simulink model "ATOM_parking_chain"  (R2026a)
settings: Solver=ode4  StopTime=100  FixedStep=0.01
StopFcn:
  | % Put every new figure in the same MATLAB Figures window as a docked tab.
  | set(groot, 'defaultFigureWindowStyle', 'docked');
  | 
  | if exist('costmap_active', 'var') && ...
  |         exist('vehicle', 'var') && ...
  |         exist('parking_path', 'var') && ...
  |         ~isempty(parking_path)
  | 
  |     plotPlan(costmap_active, vehicle, parking_path);
  | 
  | else
  | 
  |     warning('No valid parking path is available for plotting.');
  | 
  | end
  | 
  | PlotControllerReferences( ...
  |     out.controller_reference_log);
  | 
  | PlotControllerTracking( ...
  |     out.controller_tracking_log);
undefined symbols (not defined in the file): lateral, longitudinal, stanley, vehicle
(part 4 of 11)

== matlab function ATOM_parking_chain/Subsystem1/parkingNMPC ==
  settings: updateMethod=DISCRETE  sampleTime=0.04
  data: tx input; path_length output; ty input; tqz input; tqw input; tdf input; tdr input; tvx input; tax input; max_q output; X input; Y input; s_now output; ey_now output; qz input; qw input; vx input; ax_meas input; df input; dr input; x_now output; veh input; longitudinal_mode output; df_rate_cmd output; dr_rate_cmd output; nmpc_info output; segment_done output; active_segment input; endpoint_error output; a_cmd_history input; costmap input; df_ref_out output; dr_ref_out output; t_ref input; s_ref input; x_ref input; y_ref input; psi_ref input; v_ref input; a_ref input; df_nom input; dr_nom input
function [path_length, max_q, s_now, ey_now, x_now, ...
    longitudinal_mode, df_rate_cmd, dr_rate_cmd, nmpc_info, ...
    segment_done, endpoint_error, ...
    df_ref_out, dr_ref_out] = parkingNMPC( ...
    tx,ty,tqz,tqw,tdf,tdr,tvx,tax, ...
    X,Y,qz,qw,vx,ax_meas,df,dr,veh, ...
    active_segment,a_cmd_history,costmap,t_ref,s_ref,x_ref,y_ref,psi_ref,v_ref,a_ref,df_nom,dr_nom)
% Steering-only NMPC: U(:,1:2) are front/rear steering-rate commands.
% The separate parkingLongitudinalController provides acceleration.
% Both prediction loops reproduce its feedforward-plus-P law.
% Expected timing: controller/prediction 0.04 s, steering delay 0.24 s,
% acceleration delay 0.10 s. a_cmd_history is a 3-by-1 vector containing
% the actual pre-transport-delay acceleration commands, oldest first.
% This version has 13 outputs, matching the supplied Subsystem1 wiring.
persistent ref s_prev U_prev buf terminal_creep_steps
persistent previous_active_segment
persistent steering_command_state
persistent steering_alignment_pending

N  = 15;
nd = 6;

if isempty(previous_active_segment)
    previous_active_segment = active_segment;
    segment_changed = false;
else
    segment_changed = ...
        active_segment ~= previous_active_segment;

    previous_active_segment = active_segment;
end

% Build the reference during the first execution.
if isempty(ref)
    ref = buildRef( ...
    t_ref,s_ref,x_ref,y_ref,psi_ref,v_ref,a_ref, ...    
    df_nom,dr_nom);
end

if isempty(s_prev)
    s_prev = 0;
end

if isempty(U_prev)
    % Columns: front steering rate, rear steering rate
    U_prev = zeros(N,2);
end

if isempty(buf)
    % Initialize the delayed-command history from the measured wheel angles.
    buf = repmat([df, dr], nd, 1);
end

if isempty(steering_command_state)
    steering_command_state = [df,dr];
end

% History of acceleration commands already sent to the vehicle.
% Three samples are retained because the acceleration delay is 0.10 s,
% equivalent to 2.5 controller intervals at Ts = 0.04 s.
% Acceleration commands sampled externally every 0.04 seconds.
aBuf = a_cmd_history;

if isempty(terminal_creep_steps)
    terminal_creep_steps = 0.0;
end

if isempty(steering_alignment_pending)
    steering_alignment_pending = true;
end

% Rebuild the reference once when the segment changes.
if logical(segment_changed)
    ref = buildRef( ...
    t_ref,s_ref,x_ref,y_ref,psi_ref,v_ref,a_ref, ...
    df_nom,dr_nom);
    s_prev = 0;
    % Columns: front steering rate, rear steering rate
    U_prev = zeros(N,2);
    terminal_creep_steps = 0.0;
    steering_alignment_pending = true;

end
path_length = ref.s(end); max_q = max(ref.q);
[s_new, ey_now] = whereOnPath(ref, X, Y, s_prev);
s_now  = min(max(s_new, s_prev), s_prev + 0.5);   % never backwards, never a big jump forward

df_ref_out = lookupS(ref.s, ref.df, s_now);
dr_ref_out = lookupS(ref.s, ref.dr, s_now);

s_prev = s_now;

% --- the state of the car right now ---
psi   = 2*atan2(qz, qw);
x_now = [X; Y; psi; vx; df; dr; ax_meas]; %state of the nmpc controller
P     = carNumbers(veh);
M = mapNumbers(costmap);
current_collision_constraint = ...
    poseCollisionConstraint(X,Y,psi,P,M);

% Remaining path distance used by the maneuver supervisor.
d_left = max(ref.s(end) - s_now, 0);

% The segment is complete only after reaching its end and stopping.
% Actual distance from the vehicle's rear axle to the segment endpoint.
endpoint_distance = hypot( ...
    X - ref.X(end), ...
    Y - ref.Y(end));

% Heading error relative to the segment endpoint, wrapped to [-pi, pi].
heading_difference = psi - ref.psi(end);

endpoint_heading_error = atan2( ...
    sin(heading_difference), ...
    cos(heading_difference));

% ---------------- Segment arrival and stop supervision ----------------
%
% Precise tolerance:
% Used to evaluate the final tracking quality.
%
% Arrival tolerance:
% Used to decide whether the stopped vehicle may proceed to the next
% forward/reverse segment.

end_distance_tolerance = 0.05;       % [m]
end_heading_tolerance  = 2*pi/180;   % [rad]

arrive_distance_tolerance = 0.20;       % [m]
arrive_heading_tolerance = 5*pi/180;   % [rad]

stop_speed_tolerance = 0.02;         % [m/s]

% Because s_now is not allowed to decrease, end_reached remains true
% after the vehicle reaches the final path progress.
end_reached = ...
    d_left <= 0.02;

% High-accuracy endpoint condition.
pose_acceptable = ...
    (endpoint_distance <= end_distance_tolerance) && ...
    (abs(endpoint_heading_error) <= end_heading_tolerance);

% Practical condition for authorizing the next gear segment.
pose_arrived = ...
    (endpoint_distance <= arrive_distance_tolerance) && ...
    (abs(endpoint_heading_error) <= arrive_heading_tolerance);

% The vehicle must be nearly stationary before changing segments.
stopped = ...
    abs(vx) <= stop_speed_tolerance;

% Steering must be positioned for the new segment before motion begins.
steering_alignment_tolerance = 2*pi/180;

segment_start_front_steering = ref.df(1);
segment_start_rear_steering  = ref.dr(1);

front_steering_aligned = ...
    abs(df-segment_start_front_steering) <= ...
    steering_alignment_tolerance;

rear_steering_aligned = ...
    abs(dr-segment_start_rear_steering) <= ...
    steering_alignment_tolerance;

steering_aligned = ...
    front_steering_aligned && ...
    rear_steering_aligned;

% Release the alignment hold only after the measured wheels—not merely the
% requested commands—have reached the new segment's starting angles.
if steering_alignment_pending && stopped && steering_aligned
    steering_alignment_pending = false;
end

steering_alignment_active = steering_alignment_pending;

% Advance to the next segment only after reaching the endpoint progress,
% stopping, and satisfying the practical arrival tolerance.
segment_done = ...
    end_reached && ...
    stopped && ...
    pose_arrived;

% If the vehicle stops outside the arrival tolerance, keep the current
% segment active and report the failure through the controller status.
arrival_failed = ...
    end_reached && ...
    stopped && ...
    ~pose_arrived;

% Permanent endpoint diagnostics:
%   element 1: position error [m]
%   element 2: signed heading error [deg]
endpoint_error = [ ...
    endpoint_distance; ...
    endpoint_heading_error*180/pi];

% Longitudinal modes:
%   0 = follow the planned velocity profile
%   1 = slow terminal approach
%   2 = stop


longitudinal_mode = 0.0;

if steering_alignment_active

    % Keep the vehicle stopped while the wheels align.
    longitudinal_mode = 2.0;

elseif end_reached

    if pose_arrived
        % Correct endpoint pose reached.
        longitudinal_mode = 2.0;
    else
        % Continue slowly to correct the endpoint pose.
        longitudinal_mode = 1.0;
    end

end

% --- steering ---
use_nmpc = true;      % false = D1 baseline (follow the plan blindly)
% [X error, Y error, heading error, nominal steering, command change]
% Velocity/acceleration remain predicted states but have no cost terms
% in this five-weight steering objective.
w = [10, 10, 1, 0.1, 0.1];

if use_nmpc
    x0   = x_now;                                          % start from the real car
    cost = @(u) score( ...
        reshape(u,N,2), ...
        x0, ...
        s_now, ...
        buf, ...
        steering_command_state, ...
        aBuf, ...
        ref, ...
        P, ...
        w, ...
        longitudinal_mode);

    nonlinear_constraint = @(u) collisionConstraints( ...
        u, ...
        x0, ...
        s_now, ...
        buf, ...
        steering_command_state, ...
        aBuf, ...
        ref, ...
        P, ...
        M, ...
        longitudinal_mode);

    lb = -P.rateLim*ones(2*N,1);
    ub =  P.rateLim*ones(2*N,1);
    % Shared tolerance for the optimizer and the independent collision check.
    collision_tolerance = 1e-6;
    
    opts = optimoptions('fmincon', ...
        'Algorithm', 'sqp', ...
        'Display', 'none', ...
        'MaxIterations', 30, ...
        'ConstraintTolerance', collision_tolerance);
    solve_start = tic;
    
    % Optimize the front and rear steering commands.
    % Steering-angle limits are hard constraints.
    % Command changes are discouraged by the dU term in the cost function.
    [u, J_best, flag, solver_output] = fmincon( ...
        cost, U_prev(:), ...
        [], [], [], [], ...
        lb, ub, ...
        nonlinear_constraint, opts);
    
    solve_time = toc(solve_start);
    % Check whether the returned cost and commands are finite.
    finite_solution = ...
        isfinite(J_best) && ...
        all(isfinite(u));

    % Small tolerance for numerical round-off at the steering limits.
    bound_tolerance = 1e-9;

    % Check whether all optimized commands respect their bounds.
    inside_bounds = ...
        all(u >= lb - bound_tolerance) && ...
        all(u <= ub + bound_tolerance);

    % Verify the nonlinear collision constraints independently after
    % fmincon returns its candidate solution.
    collision_feasible = false;

    % Do not evaluate geometric constraints using nonfinite commands or
    % a candidate already declared invalid by the solver.
    if finite_solution && flag >= 0

        [candidate_collision_constraints,~] = ...
            collisionConstraints( ...
            u, ...
            x0, ...
            s_now, ...
            buf, ...
            steering_command_state,...
            aBuf, ...
            ref, ...
            P, ...
            M, ...
            longitudinal_mode);

        collision_feasible = ...
            all(isfinite(candidate_collision_constraints)) && ...
            all(candidate_collision_constraints <= ...
            collision_tolerance);
    end


    % Classify the optimization result.
    if ~finite_solution || ...
       ~inside_bounds || ...
       ~collision_feasible || ...
       flag < 0

        % The optimizer returned an unusable result.
        controller_status = 2;

    elseif flag == 0 || solve_time > P.controlTs

        % The result is usable, but the solver did not converge normally
        % or exceeded the controller sampling period.
        controller_status = 1;

    else

        % The solver returned a normal valid result.
        controller_status = 0;

    end

    % Endpoint-arrival diagnostics.
    % Preserve status 2 when the optimizer result itself is invalid.
    %
    % Status 5:
    %   stopped outside the 0.20 m / 5 degree arrival tolerance.
    %
    % Status 4:
    %   segment accepted using the arrival tolerance, but outside the
    %   more precise 0.05 m / 2 degree quality tolerance.
    
    if controller_status ~= 2
    
        if arrival_failed
            controller_status = 5;
    
        elseif segment_done && ~pose_acceptable
            controller_status = 4;
        end
    
    end
        
    % If the new optimizer result is unusable, verify whether the
    % remaining previous steering plan is still safe from the current
    % measured state and with the current costmap.
    fallback_collision_feasible = false;

    if controller_status == 2

        fallback_u = U_prev(:);

        fallback_finite = ...
            all(isfinite(fallback_u));

        fallback_inside_bounds = ...
            all(fallback_u >= lb - bound_tolerance) && ...
            all(fallback_u <= ub + bound_tolerance);

        if fallback_finite && fallback_inside_bounds

            [fallback_collision_constraints,~] = ...
                collisionConstraints( ...
                fallback_u, ...
                x0, ...
                s_now, ...
                buf, ...
                steering_command_state,...
                aBuf, ...
                ref, ...
                P, ...
                M, ...
                longitudinal_mode);

            fallback_collision_feasible = ...
                all(isfinite(fallback_collision_constraints)) && ...
                all(fallback_collision_constraints <= ...
                collision_tolerance);
        end
    end

    % Convert the new optimizer result into an N-by-2 steering plan.
    U_candidate = reshape(u, N, 2);
    
    % Select the steering plan that the controller is allowed to use.
    if controller_status == 2

        if fallback_collision_feasible

            % The new result is unusable, but the remaining previous
            % plan is still collision-free from the current state.
            U_selected = U_prev;

        else

            % Neither the new solution nor the previous plan is safe.
            % Request braking from the separate longitudinal controller.
            longitudinal_mode = 2.0;

            % Hold the current measured steering angles while stopping.
            % Move the desired steering command toward the measured wheel angles.
            target_front_angle = max( ...
                -P.steerMax, ...
                min(P.steerMax,df));
            
            target_rear_angle = max( ...
                -P.steerMax, ...
                min(P.steerMax,dr));
            
            hold_front_rate = ...
                (target_front_angle-steering_command_state(1))/P.controlTs;
            
            hold_rear_rate = ...
                (target_rear_angle-steering_command_state(2))/P.controlTs;
            
            hold_front_rate = max( ...
                -P.rateLim, ...
                min(P.rateLim,hold_front_rate));
            
            hold_rear_rate = max( ...
                -P.rateLim, ...
                min(P.rateLim,hold_rear_rate));
            
            U_selected = zeros(N,2);
            U_selected(1,1:2) = [hold_front_rate,hold_rear_rate];
            % Status 6 means emergency stop caused by the absence of a
            % collision-feasible steering sequence.
            controller_status = 6;
        end

    else
    
        % Status 0: normal solution.
        % Status 1: degraded but numerically valid solution.
        U_selected = U_candidate;
    
    end

    % Align the wheels directly while the vehicle is stopped at a gear change.
    % This does not move the vehicle body.
    % While steering alignment is pending, keep the vehicle stopped and do
    % not allow the NMPC steering solution to compete with the alignment.
    if steering_alignment_active

        longitudinal_mode = 2.0;
        controller_status = 7;

        % Zero rate holds the current desired steering angles while the
        % vehicle is still coming to rest.
        U_selected = zeros(N,2);

        % Begin changing the steering only after the vehicle has stopped.
        if stopped

            target_front_angle = max( ...
                -P.steerMax, ...
                min(P.steerMax,segment_start_front_steering));

            target_rear_angle = max( ...
                -P.steerMax, ...
                min(P.steerMax,segment_start_rear_steering));

            alignment_front_rate = ...
                (target_front_angle-steering_command_state(1))/P.controlTs;

            alignment_rear_rate = ...
                (target_rear_angle-steering_command_state(2))/P.controlTs;

            alignment_front_rate = max( ...
                -P.rateLim, ...
                min(P.rateLim,alignment_front_rate));

            alignment_rear_rate = max( ...
                -P.rateLim, ...
                min(P.rateLim,alignment_rear_rate));

            U_selected(1,1:2) = ...
                [alignment_front_rate,alignment_rear_rate];
        end
    end

    selected_input = U_selected(1,:);
    
    df_rate_cmd = selected_input(1);
    dr_rate_cmd = selected_input(2);
    
    selected_rate = selected_input(1:2);
    
    % Mirror the external rate-to-angle integrator inside the NMPC.
    
    sent_angle_trajectory = expandSteeringRatePlan( ...
        selected_rate,steering_command_state,P);
    
    steering_command_state = ...
        sent_angle_trajectory(end,:);
    
    updated_delay_history = ...
        [buf;sent_angle_trajectory];
    
    buf = updated_delay_history(end-nd+1:end,:);
    
    % The warm start continues to contain steering rates.
    U_prev = [U_selected(2:end,:);U_selected(end,:)];
    % Status 7 means the vehicle is intentionally stationary while its
    % measured steering aligns with the new segment.
    if steering_alignment_active && ...
            (controller_status == 0 || controller_status == 1)

        controller_status = 7;
    end

    % Status 8:
    % Terminal creep is collision-infeasible, but the stopped vehicle is
    % currently collision-free and sufficiently close to the cusp.
    % Authorize the gear change so the next segment can move away from
    % the obstacle instead of repeating an impossible creep forever.

    cusp_recovery_distance_tolerance = 0.25;        % [m]
    cusp_recovery_heading_tolerance  = 10*pi/180;   % [rad]

    safe_cusp_handoff = ...
        (controller_status == 6) && ...
        arrival_failed && ...
        ~steering_alignment_active && ...
        (current_collision_constraint <= collision_tolerance) && ...
        (endpoint_distance <= cusp_recovery_distance_tolerance) && ...
        (abs(endpoint_heading_error) <= ...
        cusp_recovery_heading_tolerance);

    if safe_cusp_handoff
        segment_done = true;
        controller_status = 8;
    end
    
    nmpc_info = [ ...
        double(J_best); ...
        double(flag); ...
        double(solve_time); ...
        double(solver_output.iterations); ...
        double(solver_output.funcCount); ...
        double(controller_status)];
    % nmpc_info = [ ...
    %     double(current_collision_constraint); ...
    %     double(flag); ...
    %     double(solve_time); ...
    %     double(solver_output.iterations); ...
    %     double(solver_output.funcCount); ...
    %     double(controller_status)];
else
    % Planner steering angles used by the non-NMPC baseline.
    target_front_angle = lookupS(ref.s,ref.df,s_now);
    target_rear_angle  = lookupS(ref.s,ref.dr,s_now);

    % Convert the required angle changes into steering-rate commands.
    df_rate_cmd = ...
        (target_front_angle-steering_command_state(1))/P.controlTs;

    dr_rate_cmd = ...
        (target_rear_angle-steering_command_state(2))/P.controlTs;

    % Apply the same steering-rate limits used by the NMPC.
    df_rate_cmd = max(-P.rateLim,min(P.rateLim,df_rate_cmd));
    dr_rate_cmd = max(-P.rateLim,min(P.rateLim,dr_rate_cmd));

    % Mirror the steering command actually selected in baseline mode.
    selected_rate = [df_rate_cmd,dr_rate_cmd];
    
    sent_angle_trajectory = expandSteeringRatePlan( ...
        selected_rate,steering_command_state,P);
    
    steering_command_state = sent_angle_trajectory(end,:);
    
    updated_delay_history = [buf;sent_angle_trajectory];
    buf = updated_delay_history(end-nd+1:end,:);
    

    U_prev = zeros(N,2);
    
    nmpc_info = [0; 0; 0; 0; 0; 3];
end
end

%--------------------------------------------------------------------------
function P = carNumbers(veh)
% All fields must be created before the structure is read.

collisionMargin = 0.5;

% Controller and internal prediction timing.
controlTs    = 0.04;
predictionTs = 0.04;

P.L        = veh(3);
P.steerMax = veh(10);
P.aMax     = veh(16);
P.rateLim  = veh(18);
P.tau      = veh(22);


%!!!!!!!!!!!!!!!!!!!!!!!!!!!!!!!!!!!!!!!!!!!!!!!!!!!!!!!!!!!!!!!!!!!!!!!!!!
P.vMax = veh(15);       % Prediction clip
P.vStateMax = veh(15);  % Explicit NMPC velocity constraint
%We have considered the maximum velocity in both the prediction and nmpc to
%be equal to the parameter's maximum value although currently it is equal
%to 50m/s!!!!!!!!!!!!!!!!!!!!!!!!!!!!!!!!!!!!!!!!!
%!!!!!!!!!!!!!!!!!!!!!!!!!!!!!!!!!!!!!!!!!!!!!!!!!!!!!!!!!!!!!!!!!!!!!!!!!!

P.controlTs = controlTs;
P.predictionTs = predictionTs;
P.substepsPerControl = round( ...
    controlTs/predictionTs);

P.accDelay = veh(19);
P.accTau   = veh(20);
P.aCmdMax  = 1.0; % Match a_cmd_limit in parkingLongitudinalController.

P.footprintMargin = collisionMargin;

P.footprintBack = ...
    -(veh(6) + collisionMargin/2);

P.footprintFront = ...
    veh(3) + veh(5) + collisionMargin/2;

P.footprintHalfWidth = ...
    (veh(4) + veh(7) + veh(8) + collisionMargin)/2;
end

%--------------------------------------------------------------------------
function M = mapNumbers(costmap)

resolution = double(costmap.info.resolution);

M.res = resolution;
M.width = double(costmap.info.width);
M.height = double(costmap.info.height);

M.originX = double(costmap.info.origin.position.x);
M.originY = double(costmap.info.origin.position.y);

M.grid = double(costmap.data)/100;

M.cellHalf = resolution/2;
end

%--------------------------------------------------------------------------
function [x1,aBuf1,df_raw,dr_raw,vx_raw] = predictStep( ...
    x0,aBuf,aCmd,dfc,drc,P)
% Predict the vehicle over one 0.04 s controller interval.

X   = x0(1);
Y   = x0(2);
psi = x0(3);
vx  = x0(4);
df  = x0(5);
dr  = x0(6);
ax  = x0(7);

%% Steering actuator

ddf = max( ...
    -P.rateLim, ...
    min(P.rateLim,(dfc-df)/P.tau));

ddr = max( ...
    -P.rateLim, ...
    min(P.rateLim,(drc-dr)/P.tau));

df_raw = df + P.predictionTs*ddf;
dr_raw = dr + P.predictionTs*ddr;

df1 = max(-P.steerMax,min(P.steerMax,df_raw));
dr1 = max(-P.steerMax,min(P.steerMax,dr_raw));

%% Acceleration delay and actuator lag

% The 0.04 s interval is divided into two 0.02 s parts.
h = 0.5*P.predictionTs;

% For a 0.10 s transport delay, the delayed command changes halfway
% through the current 0.04 s interval.
aDelayedFirst  = aBuf(1);
aDelayedSecond = aBuf(2);

% First half of the acceleration-actuator response.
axHalf = ax + ...
    h*(aDelayedFirst-ax)/P.accTau;

axHalf = max( ...
    -P.aMax, ...
    min(P.aMax,axHalf));

% Second half of the acceleration-actuator response.
ax1 = axHalf + ...
    h*(aDelayedSecond-axHalf)/P.accTau;

ax1 = max( ...
    -P.aMax, ...
    min(P.aMax,ax1));

% Integrate longitudinal acceleration over the two half-steps.
deltaVFirst = ...
    0.5*h*(ax+axHalf);

deltaVSecond = ...
    0.5*h*(axHalf+ax1);

vxFromAcceleration = ...
    vx + deltaVFirst + deltaVSecond;

% Steering changes during this controller interval, so use its
% midpoint value when predicting the vehicle motion.
dfMid = 0.5*(df+df1);
drMid = 0.5*(dr+dr1);

% Match the longitudinal-velocity equation used by Vehicle_Model.
vxMidForCoupling = ...
    0.5*(vx+vxFromAcceleration);

vehicleSpeedMid = ...
    vxMidForCoupling/max(cos(drMid),0.1);

yawRateMid = ...
    (vxMidForCoupling/P.L) * ...
    (tan(dfMid)-tan(drMid));

rearSteeringVelocityTerm = ...
    yawRateMid*vehicleSpeedMid*sin(drMid);

% Preserve the unconstrained prediction for the optimizer constraint.
vx_raw = vxFromAcceleration + ...
         P.predictionTs*rearSteeringVelocityTerm;

% Keep the numerical guard for state propagation.
vx1 = max(-P.vMax,min(P.vMax,vx_raw));

% Store the acceleration command predicted for the current cycle.
aBuf1 = [aBuf(2:end); aCmd];

%% Vehicle motion

vxMid = 0.5*(vx+vx1);

dRear = ...
    vxMid*P.predictionTs/max(cos(drMid),0.1);

[X1,Y1,psi1] = bicycleGetPose( ...
    X,Y,psi,dfMid,drMid,P.L,dRear);


x1 = [X1;Y1;psi1;vx1;df1;dr1;ax1];


end
%-------------------------------------------------------------------------
function angle_commands = expandSteeringRatePlan( ...
    rate_commands,initial_angle_command,P)

number_of_rate_commands = size(rate_commands,1);
substeps_per_command = P.substepsPerControl;

number_of_angle_samples = ...
    number_of_rate_commands*substeps_per_command;

angle_commands = zeros(number_of_angle_samples,2);

front_command = initial_angle_command(1);
rear_command  = initial_angle_command(2);

sample_index = 0;

for k = 1:number_of_rate_commands

    front_rate = max( ...
        -P.rateLim, ...
        min(P.rateLim,rate_commands(k,1)));

    rear_rate = max( ...
        -P.rateLim, ...
        min(P.rateLim,rate_commands(k,2)));

    for j = 1:substeps_per_command

        front_command = max( ...
            -P.steerMax, ...
            min(P.steerMax, ...
            front_command + ...
            P.predictionTs*front_rate));

        rear_command = max( ...
            -P.steerMax, ...
            min(P.steerMax, ...
            rear_command + ...
            P.predictionTs*rear_rate));

        sample_index = sample_index + 1;

        angle_commands(sample_index,1) = front_command;
        angle_commands(sample_index,2) = rear_command;
    end
end
end

%--------------------------------------------------------------------------
function J = score( ...
    U,x0,s0,buf,steering_command_state, ...
    aBuf,ref,P,w,longitudinal_mode)

% The two optimized inputs are front and rear steering rates.
steering_rate_plan = U(:,1:2);

candidate_angle_commands = expandSteeringRatePlan( ...
    steering_rate_plan,steering_command_state,P);

% Steering commands already waiting in the delay act first.
Ucmd = [buf;candidate_angle_commands];

x = x0;
s = s0;
J = 0;

aBufPrediction = aBuf;
modePrediction = longitudinal_mode;

% Anchor reference time at the current path progress.
t_start = lookupS(ref.s,ref.t,s0);

for k = 1:size(Ucmd,1)

    dLeftPrediction = max(ref.s(end)-s,0.0);

    if dLeftPrediction <= 0.02 && modePrediction ~= 1.0
        modePrediction = 2.0;
    end

    % Predict the external feedforward-plus-P controller at this state.
    % Use the same longitudinal prediction in collisionConstraints.
    aCmdPrediction = longitudinalCommandPrediction( ...
        ref,s,x(4),modePrediction,P);

    [x,aBufPrediction] = predictStep( ...
        x,aBufPrediction,aCmdPrediction, ...
        Ucmd(k,1),Ucmd(k,2),P);

    [s,~] = whereOnPath(ref,x(1),x(2),s);

    t_target = min( ...
        t_start + k*P.predictionTs,ref.t(end));

    X_target = lookupS(ref.t,ref.X,t_target);
    Y_target = lookupS(ref.t,ref.Y,t_target);
    psi_target = lookupS(ref.t,ref.psi,t_target);

    df_target = lookupS(ref.t,ref.df,t_target);
    dr_target = lookupS(ref.t,ref.dr,t_target);

    eX = x(1)-X_target;
    eY = x(2)-Y_target;

    dpsi = x(3)-psi_target;
    epsi = atan2(sin(dpsi),cos(dpsi));

    edf = x(5)-df_target;
    edr = x(6)-dr_target;

    J = J + ...
        w(1)*eX^2 + ...
        w(2)*eY^2 + ...
        w(3)*epsi^2 + ...
        w(4)*(edf^2 + edr^2);
end

% Penalize steering command changes.
steering_angle_changes = P.controlTs*steering_rate_plan;

J = J + w(5)*sum(steering_angle_changes(:).^2);


end

%--------------------------------------------------------------------------
function a_cmd = longitudinalCommandPrediction( ...
    ref, s, vx, longitudinal_mode, P)
% Predict the acceleration command that the separate longitudinal
% controller will generate.

Kp = 1.0;
Kp_stop = 5.0;
terminal_creep_speed = 0.05;

v_ref = lookupS(ref.s,ref.v,s);
a_ref = lookupS(ref.s,ref.a,s);

gear = ref.gear;
Kp_active = Kp;

if longitudinal_mode == 2.0

    % Stop mode.
    v_ref = 0.0;
    a_ref = 0.0;
    Kp_active = Kp_stop;

elseif longitudinal_mode == 1.0

    % Terminal-creep mode.
    v_ref = gear*terminal_creep_speed;
    a_ref = 0.0;

end

speed_error = v_ref-vx;

speed_in_gear = gear*vx;
reference_speed_in_gear = gear*v_ref;
feedforward_in_gear = gear*a_ref;

a_feedforward = a_ref;

% Apply braking feedforward only while the vehicle is moving faster
% than its reference in the intended gear direction.
if feedforward_in_gear < 0.0 && ...
        speed_in_gear <= reference_speed_in_gear

    a_feedforward = 0.0;

end

a_unsaturated = ...
    a_feedforward + Kp_active*speed_error;

a_cmd = max( ...
    -P.aCmdMax, ...
    min(P.aCmdMax,a_unsaturated));

end

%--------------------------------------------------------------------------
function v = lookupS(sv, vv, s)
% Value of vv at distance s along the route (straight line between points).
n = numel(sv);
v = vv(n);
if s <= sv(1), v = vv(1); return; end
if s >= sv(n), return; end
for i = 1:n-1
    if s <= sv(i+1)
        ds = sv(i+1) - sv(i);
        if ds < 1e-12
            v = vv(i+1);
        else
            v = vv(i) + (s - sv(i))/ds*(vv(i+1) - vv(i));
        end
        return;
    end
end
end

%--------------------------------------------------------------------------
function ref = buildRef( ...
    t_ref,s_ref,x_ref,y_ref,psi_ref,v_ref,a_ref, ...
    df_nom,dr_nom)

% Local arrays
t   = t_ref(:);
s   = s_ref(:);
Xr  = x_ref(:);
Yr  = y_ref(:);
psir = psi_ref(:);
vr  = v_ref(:);
ar  = a_ref(:);
dfr = df_nom(:);
drr = dr_nom(:);

n = numel(t);

%% Steering variation per metre

q = zeros(n,1);

for i = 1:n-1

    ds = max(s(i+1)-s(i),1e-9);

    q(i) = max( ...
        abs(dfr(i+1)-dfr(i)), ...
        abs(drr(i+1)-drr(i))) / ds;

end

if n > 1
    q(n) = q(n-1);
else
    q(1) = 0.0;
end

%% Forward or reverse gear

gear = 1;

for i = 1:n

    if abs(vr(i)) > 1e-6
        gear = sign(vr(i));
        break;
    end

end

%% Create every structure field after calculations are complete

ref.t    = t;
ref.s    = s;
ref.X    = Xr;
ref.Y    = Yr;
ref.psi  = psir;
ref.v    = vr;
ref.a    = ar;
ref.df   = dfr;
ref.dr   = drr;
ref.q    = q;
ref.gear = gear;

end

%--------------------------------------------------------------------------
function [s, ey] = whereOnPath(ref, X, Y, s_guess)
% Closest point on the route to (X,Y).
%   s  : how far along the route that point is
%   ey : how far to the side the car is (left positive)
n = numel(ref.s);
best = inf;  s = s_guess;  ey = 0;
win  = 1.5;

for pass = 1:2
    for i = 1:n-1
        if abs(ref.s(i) - s_guess) > win
            continue;
        end
        ax = ref.X(i);   ay = ref.Y(i);
        bx = ref.X(i+1); by = ref.Y(i+1);
        L2 = (bx-ax)^2 + (by-ay)^2;
        t  = ((X-ax)*(bx-ax) + (Y-ay)*(by-ay)) / max(L2, 1e-12);
        t  = min(max(t, 0), 1);
        px = ax + t*(bx-ax);   py = ay + t*(by-ay);
        d2 = (X-px)^2 + (Y-py)^2;
        if d2 < best
            best = d2;
            s  = ref.s(i) + t*(ref.s(i+1) - ref.s(i));
            ey = sign((bx-ax)*(Y-ay) - (by-ay)*(X-ax)) * sqrt(d2);
        end
    end
    if best < inf, break; end
    win = inf;
end
end

%--------------------------------------------------------------------------
function cPose = poseCollisionConstraint(X,Y,psi,P,M) %This function is added in our way for the implementation of the non-linear hard constraint of the obstacle avoidance
% Continuous collision measure for one predicted vehicle pose.
%
% fmincon convention:
%   cPose < 0  : collision-free
%   cPose = 0  : touching the obstacle or map boundary
%   cPose > 0  : collision or map-boundary violation

% Nearby obstacles begin influencing the constraint from this distance.
% This is not an additional vehicle safety margin.
influenceDistance = 1.0;

% Prevent exact geometric touching from being accepted because of
% numerical round-off.
numericalClearance = 1e-4;

ct = cos(psi);
st = sin(psi);

%% Enlarged vehicle rectangle

back = P.footprintBack;
front = P.footprintFront;
halfWidth = P.footprintHalfWidth;

vehicleCentreOffset = 0.5*(front + back);
vehicleHalfLength = 0.5*(front - back);

vehicleCentreX = X + ct*vehicleCentreOffset;
vehicleCentreY = Y + st*vehicleCentreOffset;

% Projection of the rotated vehicle rectangle onto the world axes.
vehicleProjectionX = ...
    vehicleHalfLength*abs(ct) + halfWidth*abs(st);

vehicleProjectionY = ...
    vehicleHalfLength*abs(st) + halfWidth*abs(ct);

vehicleMinX = vehicleCentreX - vehicleProjectionX;
vehicleMaxX = vehicleCentreX + vehicleProjectionX;
vehicleMinY = vehicleCentreY - vehicleProjectionY;
vehicleMaxY = vehicleCentreY + vehicleProjectionY;

%% Map-boundary constraint

mapMinX = M.originX - M.cellHalf;
mapMaxX = M.originX + (M.width-1)*M.res + M.cellHalf;

mapMinY = M.originY - M.cellHalf;
mapMaxY = M.originY + (M.height-1)*M.res + M.cellHalf;

boundaryConstraint = max( ...
    max( ...
        mapMinX - vehicleMinX, ...
        vehicleMaxX - mapMaxX), ...
    max( ...
        mapMinY - vehicleMinY, ...
        vehicleMaxY - mapMaxY));

%% Find nearby costmap cells

searchHalfX = ...
    vehicleProjectionX + M.cellHalf + influenceDistance;

searchHalfY = ...
    vehicleProjectionY + M.cellHalf + influenceDistance;

ix0 = ceil( ...
    (vehicleCentreX-searchHalfX-M.originX)/M.res);

ix1 = floor( ...
    (vehicleCentreX+searchHalfX-M.originX)/M.res);

iy0 = ceil( ...
    (vehicleCentreY-searchHalfY-M.originY)/M.res);

iy1 = floor( ...
    (vehicleCentreY+searchHalfY-M.originY)/M.res);

ix0 = max(0,ix0);
ix1 = min(M.width-1,ix1);

iy0 = max(0,iy0);
iy1 = min(M.height-1,iy1);

% A value of -influenceDistance is safely feasible.
obstacleConstraint = -influenceDistance;

% Projection of a square costmap cell onto either vehicle axis.
cellProjectionRotated = ...
    M.cellHalf*(abs(ct) + abs(st));

%% Rectangle-versus-cell constraints

if ix0 <= ix1 && iy0 <= iy1

    for iy = iy0:iy1
        for ix = ix0:ix1

            cellValue = M.grid(iy+1,ix+1);

            % Occupied cells are >= 1.
            % Unknown cells are negative and are also unsafe.
            if cellValue >= 1.0 || cellValue < 0.0

                cellX = M.originX + ix*M.res;
                cellY = M.originY + iy*M.res;

                dx = cellX - vehicleCentreX;
                dy = cellY - vehicleCentreY;

                % Overlap on the two world axes.
                overlapWorldX = ...
                    vehicleProjectionX + M.cellHalf - abs(dx);

                overlapWorldY = ...
                    vehicleProjectionY + M.cellHalf - abs(dy);

                % Cell position expressed along the vehicle axes.
                distanceLongitudinal = ct*dx + st*dy;
                distanceLateral = -st*dx + ct*dy;

                % Overlap on the two vehicle axes.
                overlapLongitudinal = ...
                    vehicleHalfLength + ...
                    cellProjectionRotated - ...
                    abs(distanceLongitudinal);

                overlapLateral = ...
                    halfWidth + ...
                    cellProjectionRotated - ...
                    abs(distanceLateral);

                % SAT collision measure for this occupied cell.
                cellConstraint = min( ...
                    min(overlapWorldX,overlapWorldY), ...
                    min(overlapLongitudinal,overlapLateral));

                obstacleConstraint = max( ...
                    obstacleConstraint, ...
                    cellConstraint);
            end
        end
    end
end

% The worst condition determines whether this pose is feasible.
cPose = ...
    max(boundaryConstraint,obstacleConstraint) + ...
    numericalClearance;
end

%--------------------------------------------------------------------------
function [c,ceq] = collisionConstraints( ...
    u,x0,s0,buf,steering_command_state, ...
    aBuf,ref,P,M,longitudinal_mode)

N = 15;

% Two optimized steering rates per prediction stage.
U = reshape(u,N,2);

steering_rate_plan = U(:,1:2);


candidate_angle_commands = expandSteeringRatePlan( ...
    steering_rate_plan,steering_command_state,P);

Ucmd = [buf;candidate_angle_commands];

numberOfPredictedSteps = size(Ucmd,1);

% One collision, four steering-angle, and two velocity inequalities.
constraints_per_step = 7;
c = zeros(constraints_per_step*numberOfPredictedSteps,1);
ceq = zeros(0,1);

x = x0;
s = s0;

aBufPrediction = aBuf;
modePrediction = longitudinal_mode;

for k = 1:numberOfPredictedSteps

    dLeftPrediction = max(ref.s(end)-s,0.0);

    if dLeftPrediction <= 0.02 && modePrediction ~= 1.0
        modePrediction = 2.0;
    end

    % Match the feedforward-plus-P prediction used by score.
    aCmdPrediction = longitudinalCommandPrediction( ...
        ref,s,x(4),modePrediction,P);

    [x,aBufPrediction,df_raw,dr_raw,vx_raw] = predictStep( ...
        x,aBufPrediction,aCmdPrediction,Ucmd(k,1),Ucmd(k,2),P);

    [s,~] = whereOnPath(ref,x(1),x(2),s);

    i = constraints_per_step*(k-1);

    c(i+1) = poseCollisionConstraint( ...
        x(1),x(2),x(3),P,M);

    c(i+2) =  df_raw-P.steerMax;
    c(i+3) = -df_raw-P.steerMax;

    c(i+4) =  dr_raw-P.steerMax;
    c(i+5) = -dr_raw-P.steerMax;
    % Hard predicted-velocity state constraint:
    % -P.vStateMax <= vx_raw <= P.vStateMax
    c(i+6) =  vx_raw - P.vStateMax;
    c(i+7) = -vx_raw - P.vStateMax;
end

end

== matlab function ATOM_parking_chain/Vehicle_Model1/Vehicle Dynamics/MATLAB Function ==
  data: state input Bus: VehicleInternalStateBus size=1; d_state output Bus: VehicleInternalStateBus size=1; command input Bus: ControlCMDBus size=1; veh input; rear_steering_command input
function d_state = vehicleDynamics(state, command, veh, rear_steering_command)

%%%%%%%%%%%%%%%%%%%%%%%%%%%%%%%%%%%%%%
%%%%%%%%%%%%%%%%%%%%%%%%%%%%%%%%%%%%%%
% Description:
% This vehicleDynamics model follows DELAY_STEER_ACC_GEARED
% model, it doesn't presents a model for gear management
% since its not something we're going to modify on Autoware for 4WS
% implementation.
%
% Inputs:
% - state: VehicleInternalStateBus. It contains the state of the vehicle
%          at time instant t. 
% - command: /control/command/control_cmd topic --> ControlCMDBus.
%          It contains the desired acc and steering commands coming from
%          the control region.
%
% - Parameters
% - vehicle: vehicle parameters struct defined in vehicleParameters.m.

% Outputs: 
% - d_state: It contains the derivative of the state of the vehicle at time
%          instant t+1.
%%%%%%%%%%%%%%%%%%%%%%%%%%%%%%%%%%%%%%
%%%%%%%%%%%%%%%%%%%%%%%%%%%%%%%%%%%%%%


% inside MATLAB Function: input is veh_in (1xN double)
v = veh; % 1xN numeric row

vehicle.param.wheel_radius    = v(1);
vehicle.param.wheel_width     = v(2);
vehicle.param.wheel_base      = v(3);
vehicle.param.wheel_tread     = v(4);
vehicle.param.front_overhang  = v(5);
vehicle.param.rear_overhang   = v(6);
vehicle.param.left_overhang   = v(7);
vehicle.param.right_overhang  = v(8);
vehicle.param.vehicle_height  = v(9);
vehicle.param.max_steer_angle = v(10);

% decode integer-coded enums (example)
vehicle.sim.vehicle_model_type = int32(v(11));    % or map to strings if needed
vehicle.sim.initialize_source  = int32(v(12));

vehicle.sim.timer_sampling_time_ms = v(13);
vehicle.sim.add_measurement_noise = logical(v(14));
vehicle.sim.vel_lim        = v(15);
vehicle.sim.vel_rate_lim   = v(16);
vehicle.sim.steer_lim      = v(17);
vehicle.sim.steer_rate_lim = v(18);
vehicle.sim.acc_time_delay = v(19);
vehicle.sim.acc_time_constant = v(20);
vehicle.sim.steer_time_delay   = v(21);
vehicle.sim.steer_time_constant= v(22);
vehicle.sim.x_stddev = v(23);
vehicle.sim.y_stddev = v(24);
vehicle.sim.steer_dead_band = v(25);
vehicle.sim.steer_bias = v(26);
vehicle.sim.debug_acc_scaling_factor = v(27);
vehicle.sim.debug_steer_scaling_factor = v(28);

% Parameter for 4WS
vehicle.param.rear_steering_ratio = veh(29);
rear_steering_ratio = vehicle.param.rear_steering_ratio;

%% ==========================
% Saturation function
% ===========================

sat = @(val, upper, lower) min(max(val,lower),upper);



%% ==========================
% Current state
% ===========================

vx = sat( ...
    state.vx,...
    vehicle.sim.vel_lim,...
   -vehicle.sim.vel_lim);


acc = sat( ...
    state.acc,...
    vehicle.sim.vel_rate_lim,...
   -vehicle.sim.vel_rate_lim);


yaw = state.yaw;

steer_front = state.steer_front;
steer_rear = state.steer_rear;          % Modified for 4WS  


%% ==========================
% Input commands
% ===========================

acc_des = sat( ...
    command.longitudinal.acceleration,...
    vehicle.sim.vel_rate_lim,...
   -vehicle.sim.vel_rate_lim);


acc_des = acc_des * ...
    vehicle.sim.debug_acc_scaling_factor;



steer_front_des = sat( ...
    command.lateral.steering_tire_angle,...
    vehicle.sim.steer_lim,...
   -vehicle.sim.steer_lim);


steer_front_des = steer_front_des * ...
    vehicle.sim.debug_steer_scaling_factor;

steer_rear_des = sat( ...                                            % Modified for 4WS
    rear_steering_command,...
    vehicle.sim.steer_lim,...
    -vehicle.sim.steer_lim);


steer_rear_des = steer_rear_des * ...                                % Modified for 4WS
    vehicle.sim.debug_steer_scaling_factor;



%% ==========================
% Steering dynamics
% ===========================

% getSteer() in simple_planning_simulator corresponds to state.steer
% From the phisical vehicle front_steer and rear_steer are measured.

steer_diff_front = steer_front - steer_front_des;

steer_diff_rear = steer_rear  - steer_rear_des;             % Modified for 4WS


% dead band

if steer_diff_front > vehicle.sim.steer_dead_band

    steer_diff_with_dead_band_front = ...
        steer_diff_front - vehicle.sim.steer_dead_band;


elseif steer_diff_front < -vehicle.sim.steer_dead_band

    steer_diff_with_dead_band_front = ...
        steer_diff_front + vehicle.sim.steer_dead_band;


else

    steer_diff_with_dead_band_front = 0;

end



if steer_diff_rear > vehicle.sim.steer_dead_band            % Modified for 4WS

    steer_diff_with_dead_band_rear = ...
        steer_diff_rear - vehicle.sim.steer_dead_band;


elseif steer_diff_rear < -vehicle.sim.steer_dead_band

    steer_diff_with_dead_band_rear = ...
        steer_diff_rear + vehicle.sim.steer_dead_band;


else

    steer_diff_with_dead_band_rear = 0;

end



steer_rate_front = sat( ...
    -steer_diff_with_dead_band_front / vehicle.sim.steer_time_constant,...
     vehicle.sim.steer_rate_lim,...
    -vehicle.sim.steer_rate_lim);

steer_rate_rear = sat( ...                                                  % Modified for 4WS
    -steer_diff_with_dead_band_rear / vehicle.sim.steer_time_constant,...
    vehicle.sim.steer_rate_lim,...
    -vehicle.sim.steer_rate_lim);



%% ==========================
% State derivative
% ===========================

%--------------------------------------------------------------
% 4WS kinematic bicycle model
%
% Assumptions:
%   - Pure rolling
%   - alpha_f = alpha_r = 0
%   - No tire dynamics
%   - No lateral slip dynamics
%
% beta is the geometric vehicle sideslip angle. Since Autoware defines
% reference frame of the vehicle equal to centre of the rear axle, then
% beta = steer_rear
%--------------------------------------------------------------

L = vehicle.param.wheel_base;


beta = steer_rear;                              % Modified for 4WS


vel = vx/cos(beta);                             % Modified for 4WS


yaw_rate = ...                                  % Modified for 4WS
    (vx/L) * ...
    (tan(steer_front)-tan(steer_rear));


d_state.x = vel*cos(yaw + beta);                % Modified for 4WS

d_state.y = vel*sin(yaw + beta);                % Modified for 4WS


d_state.yaw = yaw_rate;                         % Modified for 4WS


d_state.vx = acc + yaw_rate*vel*sin(beta);


d_state.steer_front = steer_rate_front;

d_state.steer_rear = steer_rate_rear;           % Modified for 4WS

d_state.acc = ...
    -(acc-acc_des)/vehicle.sim.acc_time_constant;

end

== matlab function ATOM_parking_chain/Vehicle_Model1/localization//acceleration function ==
  data: state input Bus: VehicleInternalStateBus; accel output Bus: AccelerationBus; veh input
function accel = IntStateToAccelerationState(state,veh)

L = veh(3);

vx = state.vx;
ax = state.acc;

delta_f = state.steer_front;
delta_r = state.steer_rear;

yaw_rate = (vx/L)*(tan(delta_f)-tan(delta_r));

ay = vx*yaw_rate;

accel.acceleration.linear.x = ax;
accel.acceleration.linear.y = ay;
accel.acceleration.linear.z = 0;

accel.acceleration.angular.x = 0;
accel.acceleration.angular.y = 0;
accel.acceleration.angular.z = 0;

end

== matlab function ATOM_parking_chain/Vehicle_Model1/localization//kinematic_state function ==
  data: state input Bus: VehicleInternalStateBus; kinematic output Bus: KinematicStateBus; veh input
function kinematic = IntStateToKinematicState(state, veh)


%% Vehicle parameters

L = veh(3);


%% Current state

x = state.x;
y = state.y;
yaw = state.yaw;



% NOTE:
% vx is the longitudinal velocity expressed in the vehicle body frame
% (base_link located at the center of the rear axle).
% The vehicle speed magnitude is reconstructed as
%
%   v = vx / cos(delta_r)
%
% under the pure-rolling assumption (alpha_f = alpha_r = 0).

vx = state.vx;

steer_front = state.steer_front;
steer_rear  = state.steer_rear;


%% Pose

kinematic.pose.position.x = x;
kinematic.pose.position.y = y;
kinematic.pose.position.z = 0;


[qx,qy,qz,qw] = yawToQuaternion(yaw);

% quaternion from yaw only

kinematic.pose.orientation.x = qx;
kinematic.pose.orientation.y = qy;
kinematic.pose.orientation.z = qz;
kinematic.pose.orientation.w = qw;



%% Twist

% Body frame velocity

kinematic.twist.linear.x = vx;

kinematic.twist.linear.y = ...              % Modified for 4WS considering beta = steer_rear
    vx*tan(steer_rear);

kinematic.twist.linear.z = 0;



% Angular velocity

kinematic.twist.angular.x = 0;
kinematic.twist.angular.y = 0;

kinematic.twist.angular.z = ...
    (vx/L) * ...
    (tan(steer_front)-tan(steer_rear));


end
